simulink model "hfi_flux_split_pmsm"  (R2026a)
settings: Solver=FixedStepDiscrete  StartTime=0  StopTime=16.0  FixedStep=1/15000
PreLoadFcn:
  | addpath('F:\code\foc\Doc\matlab');
StartFcn:
  | clear sl_split_command sl_split_angle_manager sl_split_speed_pi sl_split_speed_pi_stable sl_split_fw sl_split_duty_calc sl_split_duty_lpf sl_split_fw_duty_map sl_split_fw_backoff sl_split_fw_ramp sl_split_current_circle sl_split_hfi_observer_sync sl_split_angle_errors sl_split_encoder_feedback sl_split_hall_feedback sl_split_feedback_select sl_split_current_pi sl_hfi sl_flux sl_pmsm_discrete;
settings Model: Creator=15403  LastModifiedBy=15403

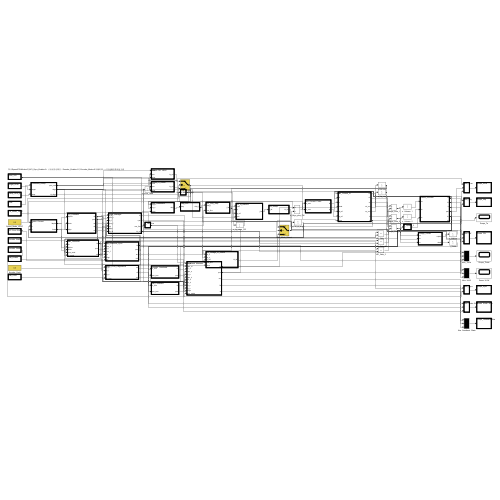
[thumbnail: Simulink's stored preview of the top-level diagram]
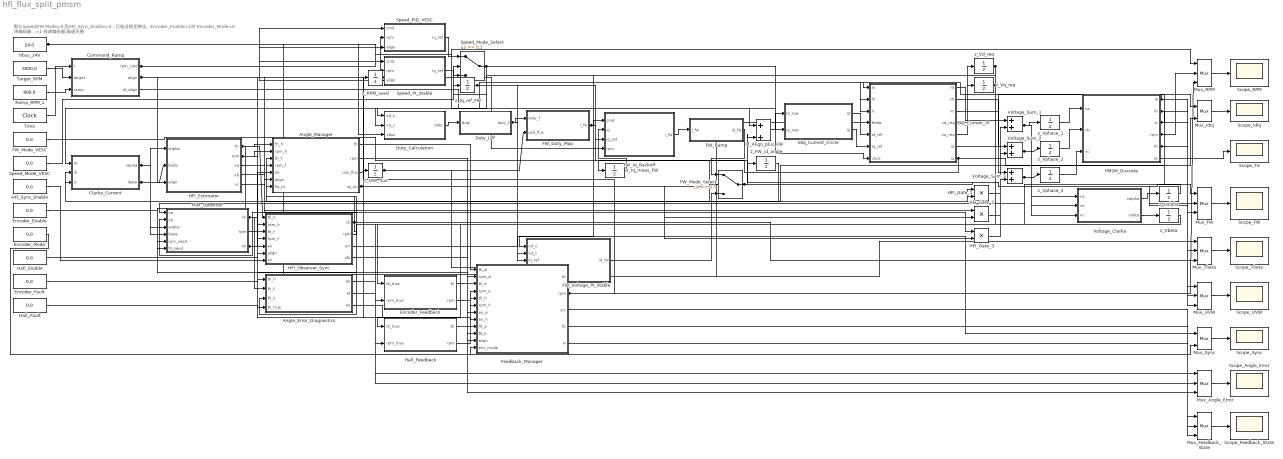
== system hfi_flux_split_pmsm ==
  note: 默认Speed/FW Mode=0且HFI_Sync_Enable=0：已验证稳定路径。Encoder_Enable=1时 Encoder_Mode=0 纯编码器，=1 低速编码器/高速无感
  Angle_Error_Diagnostics : MATLAB Function  TreatAsAtomicUnit=on
  Angle_Manager : MATLAB Function  TreatAsAtomicUnit=on
  Clarke_Current : MATLAB Function  TreatAsAtomicUnit=on
  Command_Ramp : MATLAB Function  TreatAsAtomicUnit=on
  DQ_Current_PI : MATLAB Function  TreatAsAtomicUnit=on
  Duty_Calculation : MATLAB Function  TreatAsAtomicUnit=on
  Duty_LPF : MATLAB Function  TreatAsAtomicUnit=on
  Encoder_Enable : Constant  Value=0.0
  Encoder_Fault : Constant  Value=0.0
  Encoder_Feedback : MATLAB Function  TreatAsAtomicUnit=on
  Encoder_Mode : Constant  Value=0.0
  FW_Duty_Map : MATLAB Function  TreatAsAtomicUnit=on
  FW_Iq_Backoff : MATLAB Function  TreatAsAtomicUnit=on
  FW_Mode_Select : Switch  Threshold=0.5  SaturateOnIntegerOverflow=off  InputSameDT=off
  FW_Mode_VESC : Constant  Value=0.0
  FW_Ramp : MATLAB Function  TreatAsAtomicUnit=on
  FW_Voltage_PI_Stable : MATLAB Function  TreatAsAtomicUnit=on
  Feedback_Manager : MATLAB Function  TreatAsAtomicUnit=on
  Flux_Observer : MATLAB Function  TreatAsAtomicUnit=on
  HFI_Estimator : MATLAB Function  TreatAsAtomicUnit=on
  HFI_Gate_1 : Product
  HFI_Gate_2 : Product
  HFI_Gate_3 : Product
  HFI_Observer_Sync : MATLAB Function  TreatAsAtomicUnit=on
  HFI_Sync_Enable : Constant  Value=0.0
  Hall_Enable : Constant  Value=0.0
  Hall_Fault : Constant  Value=0.0
  Hall_Feedback : MATLAB Function  TreatAsAtomicUnit=on
  IdIq_Current_Circle : MATLAB Function  TreatAsAtomicUnit=on
  Id_Align_plus_FW : Sum
  Mux_Angle_Error : Mux  Inputs=3
  Mux_FW : Mux  Inputs=3
  Mux_Feedback_State : Mux  Inputs=3
  Mux_IdIq : Mux  Inputs=2
  Mux_RPM : Mux  Inputs=3
  Mux_Sync : Mux  Inputs=2
  Mux_Theta : Mux  Inputs=3
  Mux_UVW : Mux  Inputs=3
  PMSM_Discrete : MATLAB Function  TreatAsAtomicUnit=on
  Ramp_RPM_s : Constant  Value=800.0
  Scope_Angle_Error : Scope
  Scope_FW : Scope
  Scope_Feedback_State : Scope
  Scope_IdIq : Scope
  Scope_RPM : Scope
  Scope_Sync : Scope
  Scope_Te : Scope
  Scope_Theta : Scope
  Scope_UVW : Scope
  Speed_Mode_Select : Switch  Threshold=0.5  SaturateOnIntegerOverflow=off  InputSameDT=off
  Speed_Mode_VESC : Constant  Value=0.0
  Speed_PID_VESC : MATLAB Function  TreatAsAtomicUnit=on
  Speed_PI_Stable : MATLAB Function  TreatAsAtomicUnit=on
  Target_RPM : Constant  Value=3000.0
  Time : DigitalClock  SampleTime=1/15000
  Vbus_24V : Constant  Value=24.0
  Voltage_Clarke : MATLAB Function  TreatAsAtomicUnit=on
  Voltage_Sum_1 : Sum
  Voltage_Sum_2 : Sum
  Voltage_Sum_3 : Sum
  z_FW_id_angle : UnitDelay  SampleTime=1/15000
  z_Iq_meas_FW : UnitDelay  SampleTime=1/15000
  z_Iq_ref_FW : UnitDelay  SampleTime=1/15000
  z_RPM_used : UnitDelay  SampleTime=1/15000
  z_Use_flux : UnitDelay  SampleTime=1/15000
  z_Valpha : UnitDelay  SampleTime=1/15000
  z_Vbeta : UnitDelay  SampleTime=1/15000
  z_Vd_req : UnitDelay  SampleTime=1/15000
  z_Vphase_1 : UnitDelay  SampleTime=1/15000
  z_Vphase_2 : UnitDelay  SampleTime=1/15000
  z_Vphase_3 : UnitDelay  SampleTime=1/15000
  z_Vq_req : UnitDelay  SampleTime=1/15000
  wires:
  Time/1 -> Command_Ramp/1(t)
  Target_RPM/1 -> Command_Ramp/2(target)
  Ramp_RPM_s/1 -> Command_Ramp/3(ramp)
  PMSM_Discrete/1(ia) -> Clarke_Current/1(ia), DQ_Current_PI/1(ia), Mux_UVW/1
  PMSM_Discrete/2(ib) -> Clarke_Current/2(ib), DQ_Current_PI/2(ib), Mux_UVW/2
  PMSM_Discrete/3(ic) -> Clarke_Current/3(ic), DQ_Current_PI/3(ic), Mux_UVW/3
  Clarke_Current/1(ialpha) -> HFI_Estimator/1(ialpha), Flux_Observer/3(ialpha)
  Clarke_Current/2(ibeta) -> HFI_Estimator/2(ibeta), Flux_Observer/4(ibeta)
  Command_Ramp/2(align) -> HFI_Estimator/3(align), HFI_Observer_Sync/6(align), Angle_Manager/6(align), Feedback_Manager/11(align), Speed_PI_Stable/3(align), Speed_PID_VESC/3(align)
  z_Valpha/1 -> Flux_Observer/1(va)
  z_Vbeta/1 -> Flux_Observer/2(vb)
  HFI_Estimator/2(rpm) -> Flux_Observer/5(rpm_seed), HFI_Observer_Sync/2(rpm_h), Angle_Manager/2(rpm_h)
  HFI_Estimator/1(th) -> Flux_Observer/6(th_seed), HFI_Observer_Sync/1(th_h), Angle_Error_Diagnostics/1(th_h), Angle_Manager/1(th_h)
  Flux_Observer/1(th) -> HFI_Observer_Sync/3(th_f), Angle_Error_Diagnostics/2(th_f)
  Flux_Observer/2(rpm) -> HFI_Observer_Sync/4(rpm_f)
  Flux_Observer/3(ok) -> HFI_Observer_Sync/5(ok), Angle_Manager/5(ok)
  HFI_Sync_Enable/1 -> HFI_Observer_Sync/7(en)
  HFI_Observer_Sync/1(th) -> Angle_Error_Diagnostics/3(th_s), Angle_Manager/3(th_f), Mux_Theta/3
  PMSM_Discrete/5(th) -> Angle_Error_Diagnostics/4(th_true), Encoder_Feedback/1(th_true), Hall_Feedback/1(th_true), Mux_Theta/2
  HFI_Observer_Sync/2(rpm) -> Angle_Manager/4(rpm_f)
  FW_Mode_Select/1 -> z_FW_id_angle/1, Id_Align_plus_FW/2, Mux_FW/3
  z_FW_id_angle/1 -> Angle_Manager/7(fw_id)
  PMSM_Discrete/4(rpm) -> Encoder_Feedback/2(rpm_true), Hall_Feedback/2(rpm_true), Mux_RPM/2
  Angle_Manager/1(th) -> Feedback_Manager/1(th_sl)
  Angle_Manager/2(rpm) -> Feedback_Manager/2(rpm_sl)
  Encoder_Feedback/1(th) -> Feedback_Manager/3(th_e)
  Encoder_Feedback/2(rpm) -> Feedback_Manager/4(rpm_e)
  Hall_Feedback/1(th) -> Feedback_Manager/5(th_h)
  Hall_Feedback/2(rpm) -> Feedback_Manager/6(rpm_h)
  Encoder_Enable/1 -> Feedback_Manager/7(en_e)
  Hall_Enable/1 -> Feedback_Manager/8(en_h)
  Encoder_Fault/1 -> Feedback_Manager/9(flt_e)
  Hall_Fault/1 -> Feedback_Manager/10(flt_h)
  Encoder_Mode/1 -> Feedback_Manager/12(enc_mode)
  Command_Ramp/1(rpm_cmd) -> Speed_PI_Stable/1(cmd), Speed_PID_VESC/1(cmd), Mux_RPM/1
  Feedback_Manager/2(rpm) -> z_RPM_used/1, Mux_RPM/3
  z_RPM_used/1 -> Speed_PI_Stable/2(rpm), Speed_PID_VESC/2(rpm), FW_Iq_Backoff/4(rpm)
  Speed_PID_VESC/1(iq_ref) -> Speed_Mode_Select/1
  Speed_Mode_VESC/1 -> Speed_Mode_Select/2
  Speed_PI_Stable/1(iq_ref) -> Speed_Mode_Select/3
  z_Vd_req/1 -> Duty_Calculation/1(vd_z), FW_Voltage_PI_Stable/1(vd_z)
  z_Vq_req/1 -> Duty_Calculation/2(vq_z), FW_Voltage_PI_Stable/2(vq_z)
  Vbus_24V/1 -> Duty_Calculation/3(vbus), FW_Voltage_PI_Stable/5(vbus), DQ_Current_PI/7(vbus)
  Duty_Calculation/1(duty) -> Duty_LPF/1(duty)
  Duty_LPF/1(duty_f) -> FW_Duty_Map/1(duty_f), Mux_FW/1
  Speed_Mode_Select/1 -> z_Iq_ref_FW/1, IdIq_Current_Circle/2(iq_raw)
  Angle_Manager/3(use_flux) -> z_Use_flux/1
  z_Use_flux/1 -> FW_Duty_Map/2(use_flux), FW_Voltage_PI_Stable/4(use_flux)
  FW_Duty_Map/1(i_fw) -> FW_Iq_Backoff/1(cmd), Mux_FW/2
  z_Iq_meas_FW/1 -> FW_Iq_Backoff/2(iq)
  z_Iq_ref_FW/1 -> FW_Iq_Backoff/3(iq_ref), FW_Voltage_PI_Stable/3(iq_ref)
  FW_Iq_Backoff/1(i_fw) -> FW_Ramp/1(i_fw)
  FW_Ramp/1(id_fw) -> FW_Mode_Select/1
  FW_Mode_VESC/1 -> FW_Mode_Select/2
  FW_Voltage_PI_Stable/1(id_fw) -> FW_Mode_Select/3
  Command_Ramp/3(id_align) -> Id_Align_plus_FW/1
  Id_Align_plus_FW/1 -> IdIq_Current_Circle/1(id_raw)
  Feedback_Manager/1(th) -> DQ_Current_PI/4(theta), Mux_Theta/1
  IdIq_Current_Circle/1(id) -> DQ_Current_PI/5(id_ref)
  IdIq_Current_Circle/2(iq) -> DQ_Current_PI/6(iq_ref)
  DQ_Current_PI/4(vd_req) -> z_Vd_req/1
  DQ_Current_PI/5(vq_req) -> z_Vq_req/1
  DQ_Current_PI/7(iq) -> z_Iq_meas_FW/1, Mux_IdIq/2
  HFI_Estimator/3(va) -> HFI_Gate_1/1
  Angle_Manager/4(inj_on) -> HFI_Gate_1/2, HFI_Gate_2/2, HFI_Gate_3/2
  DQ_Current_PI/1(va) -> Voltage_Sum_1/1
  HFI_Gate_1/1 -> Voltage_Sum_1/2
  Voltage_Sum_1/1 -> z_Vphase_1/1, Voltage_Clarke/1(va)
  z_Vphase_1/1 -> PMSM_Discrete/1(va)
  HFI_Estimator/4(vb) -> HFI_Gate_2/1
  DQ_Current_PI/2(vb) -> Voltage_Sum_2/1
  HFI_Gate_2/1 -> Voltage_Sum_2/2
  Voltage_Sum_2/1 -> z_Vphase_2/1, Voltage_Clarke/2(vb)
  z_Vphase_2/1 -> PMSM_Discrete/2(vb)
  HFI_Estimator/5(vc) -> HFI_Gate_3/1
  DQ_Current_PI/3(vc) -> Voltage_Sum_3/1
  HFI_Gate_3/1 -> Voltage_Sum_3/2
  Voltage_Sum_3/1 -> z_Vphase_3/1, Voltage_Clarke/3(vc)
  z_Vphase_3/1 -> PMSM_Discrete/3(vc)
  Voltage_Clarke/1(valpha) -> z_Valpha/1
  Voltage_Clarke/2(vbeta) -> z_Vbeta/1
  Mux_RPM/1 -> Scope_RPM/1
  DQ_Current_PI/6(id) -> Mux_IdIq/1
  Mux_IdIq/1 -> Scope_IdIq/1
  PMSM_Discrete/6(te) -> Scope_Te/1
  Mux_FW/1 -> Scope_FW/1
  Mux_Theta/1 -> Scope_Theta/1
  Mux_UVW/1 -> Scope_UVW/1
  HFI_Observer_Sync/3(err) -> Mux_Sync/1
  HFI_Observer_Sync/4(ofs) -> Mux_Sync/2
  Mux_Sync/1 -> Scope_Sync/1
  Angle_Error_Diagnostics/1(eh) -> Mux_Angle_Error/1
  Angle_Error_Diagnostics/2(ef) -> Mux_Angle_Error/2
  Angle_Error_Diagnostics/3(es) -> Mux_Angle_Error/3
  Mux_Angle_Error/1 -> Scope_Angle_Error/1
  Feedback_Manager/3(src) -> Mux_Feedback_State/1
  Feedback_Manager/4(fb) -> Mux_Feedback_State/2
  Feedback_Manager/5(w) -> Mux_Feedback_State/3
  Mux_Feedback_State/1 -> Scope_Feedback_State/1

== matlab function hfi_flux_split_pmsm/Encoder_Feedback ==
  data: th_true input; th output; rpm_true input; rpm output
function [th,rpm]=fcn(th_true,rpm_true)              
                                                    [th,rpm]=sl_split_encoder_feedback(th_true,rpm_true);
                                                    end

== matlab function hfi_flux_split_pmsm/Hall_Feedback ==
  data: th_true input; th output; rpm_true input; rpm output
function [th,rpm]=fcn(th_true,rpm_true)           
                                                 [th,rpm]=sl_split_hall_feedback(th_true,rpm_true);
                                                 end

== matlab function hfi_flux_split_pmsm/Feedback_Manager ==
  data: th_sl input; th output; rpm_sl input; th_e input; rpm_e input; th_h input; rpm_h input; en_e input; en_h input; flt_e input; flt_h input; align input; enc_mode input; rpm output; src output; fb output; w output
function [th,rpm,src,fb,w]=fcn(th_sl,rpm_sl,th_e,rpm_e,th_h,rpm_h,en_e,en_h,flt_e,flt_h,align,enc_mode)             
                                                                                                                   [th,rpm,src,fb,w]=sl_split_feedback_select(th_sl,rpm_sl,th_e,rpm_e,th_h,rpm_h,en_e,en_h,flt_e,flt_h,align,enc_mode);
                                                                                                                   end

== matlab function hfi_flux_split_pmsm/Speed_PI_Stable ==
  data: cmd input; iq_ref output; rpm input; align input
function iq_ref=fcn(cmd,rpm,align)             
                                              iq_ref=sl_split_speed_pi_stable(cmd,rpm,align);
                                              end

== matlab function hfi_flux_split_pmsm/Speed_PID_VESC ==
  data: cmd input; iq_ref output; rpm input; align input
function iq_ref=fcn(cmd,rpm,align)      
                                       iq_ref=sl_split_speed_pi(cmd,rpm,align);
                                       end

== matlab function hfi_flux_split_pmsm/Duty_Calculation ==
  data: vd_z input; duty output; vq_z input; vbus input
function duty=fcn(vd_z,vq_z,vbus)       
                                       duty=sl_split_duty_calc(vd_z,vq_z,vbus);
                                       end

== matlab function hfi_flux_split_pmsm/Duty_LPF ==
  data: duty input; duty_f output
function duty_f=fcn(duty)      
                              duty_f=sl_split_duty_lpf(duty);
                              end

== matlab function hfi_flux_split_pmsm/FW_Duty_Map ==
  data: duty_f input; i_fw output; use_flux input
function i_fw=fcn(duty_f,use_flux)         
                                          i_fw=sl_split_fw_duty_map(duty_f,use_flux);
                                          end

== matlab function hfi_flux_split_pmsm/FW_Iq_Backoff ==
  data: cmd input; i_fw output; iq input; iq_ref input; rpm input
function i_fw=fcn(cmd,iq,iq_ref,rpm)        
                                           i_fw=sl_split_fw_backoff(cmd,iq,iq_ref,rpm);
                                           end

== matlab function hfi_flux_split_pmsm/FW_Ramp ==
  data: i_fw input; id_fw output
function id_fw=fcn(i_fw)     
                            id_fw=sl_split_fw_ramp(i_fw);
                            end

== matlab function hfi_flux_split_pmsm/FW_Voltage_PI_Stable ==
  data: vd_z input; id_fw output; vq_z input; iq_ref input; use_flux input; vbus input
function id_fw=fcn(vd_z,vq_z,iq_ref,use_flux,vbus)
                                                 id_fw=sl_split_fw(vd_z,vq_z,iq_ref,use_flux,vbus);
                                                 end

== matlab function hfi_flux_split_pmsm/Clarke_Current ==
  data: ia input; ialpha output; ib input; ic input; ibeta output
function [ialpha,ibeta]=fcn(ia,ib,ic)
                                    [ialpha,ibeta]=foc.clarke(ia,ib,ic); 
                                    end

== matlab function hfi_flux_split_pmsm/IdIq_Current_Circle ==
  data: id_raw input; id output; iq_raw input; iq output
function [id,iq]=fcn(id_raw,iq_raw)            
                                              [id,iq]=sl_split_current_circle(id_raw,iq_raw);
                                              end

== matlab function hfi_flux_split_pmsm/DQ_Current_PI ==
  data: ia input; va output; ib input; ic input; theta input; id_ref input; iq_ref input; vbus input; vb output; vc output; vd_req output; vq_req output; id output; iq output
function [va,vb,vc,vd_req,vq_req,id,iq]=fcn(ia,ib,ic,theta,id_ref,iq_ref,vbus)        
                                                                                     [va,vb,vc,vd_req,vq_req,id,iq]=sl_split_current_pi(ia,ib,ic,theta,id_ref,iq_ref,vbus);
                                                                                     end

== matlab function hfi_flux_split_pmsm/Voltage_Clarke ==
  data: va input; valpha output; vb input; vc input; vbeta output
function [valpha,vbeta]=fcn(va,vb,vc)
                                    [valpha,vbeta]=foc.clarke(va,vb,vc); 
                                    end

== matlab function hfi_flux_split_pmsm/PMSM_Discrete ==
  data: va input; ia output; vb input; vc input; ib output; ic output; rpm output; th output; te output
function [ia,ib,ic,rpm,th,te]=fcn(va,vb,vc)     
                                               [ia,ib,ic,rpm,th,te]=sl_pmsm_discrete(va,vb,vc);
                                               end

== matlab function hfi_flux_split_pmsm/Command_Ramp ==
  data: t input; rpm_cmd output; target input; ramp input; align output; id_align output
function [rpm_cmd,align,id_align]=fcn(t,target,ramp)     
                                                        [rpm_cmd,align,id_align]=sl_split_command(t,target,ramp);
                                                        end

== matlab function hfi_flux_split_pmsm/HFI_Estimator ==
  data: ialpha input; th output; ibeta input; align input; rpm output; va output; vb output; vc output
function [th,rpm,va,vb,vc]=fcn(ialpha,ibeta,align)
                                                 [th,rpm,va,vb,vc]=sl_hfi(ialpha,ibeta,0.0,align); 
                                                 end

== matlab function hfi_flux_split_pmsm/Flux_Observer ==
  data: va input; th output; vb input; ialpha input; ibeta input; rpm_seed input; th_seed input; rpm output; ok output
function [th,rpm,ok]=fcn(va,vb,ialpha,ibeta,rpm_seed,th_seed)
                                                            [th,rpm,ok]=sl_flux(va,vb,ialpha,ibeta,rpm_seed,th_seed);    
                                                            end

== matlab function hfi_flux_split_pmsm/HFI_Observer_Sync ==
  data: th_h input; th output; rpm_h input; th_f input; rpm_f input; ok input; align input; en input; rpm output; err output; ofs output
function [th,rpm,err,ofs]=fcn(th_h,rpm_h,th_f,rpm_f,ok,align,en)               
                                                                              [th,rpm,err,ofs]=sl_split_hfi_observer_sync(th_h,rpm_h,th_f,rpm_f,ok,align,en);
                                                                              end

== matlab function hfi_flux_split_pmsm/Angle_Error_Diagnostics ==
  data: th_h input; eh output; th_f input; th_s input; th_true input; ef output; es output
function [eh,ef,es]=fcn(th_h,th_f,th_s,th_true)          
                                                        [eh,ef,es]=sl_split_angle_errors(th_h,th_f,th_s,th_true);
                                                        end

== matlab function hfi_flux_split_pmsm/Angle_Manager ==
  data: th_h input; th output; rpm_h input; th_f input; rpm_f input; ok input; align input; fw_id input; rpm output; use_flux output; inj_on output
function [th,rpm,use_flux,inj_on]=fcn(th_h,rpm_h,th_f,rpm_f,ok,align,fw_id)           
                                                                                     [th,rpm,use_flux,inj_on]=sl_split_angle_manager(th_h,rpm_h,th_f,rpm_f,ok,align,fw_id);
                                                                                     end
